simulink model "CHBPWM"  (R2022a)
settings: Solver=ode23  StartTime=0.0  StopTime=0.1  MaxStep=1e-5  RelTol=1e-3
libraries: spsDCVoltageSourceLib x1, spsThreePhaseSeriesRLCBranchLib x1, spsThreePhaseVIMeasurementLib x1, spsUniversalBridgeLib x1, spspowerguiLib x1
settings Model: Creator=123  LastModifiedBy=123

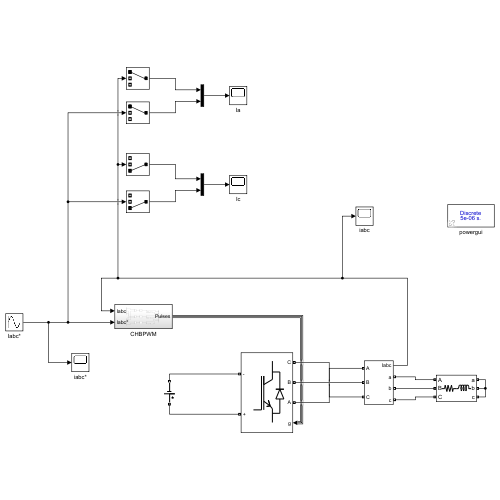
[thumbnail: Simulink's stored preview of the top-level diagram]
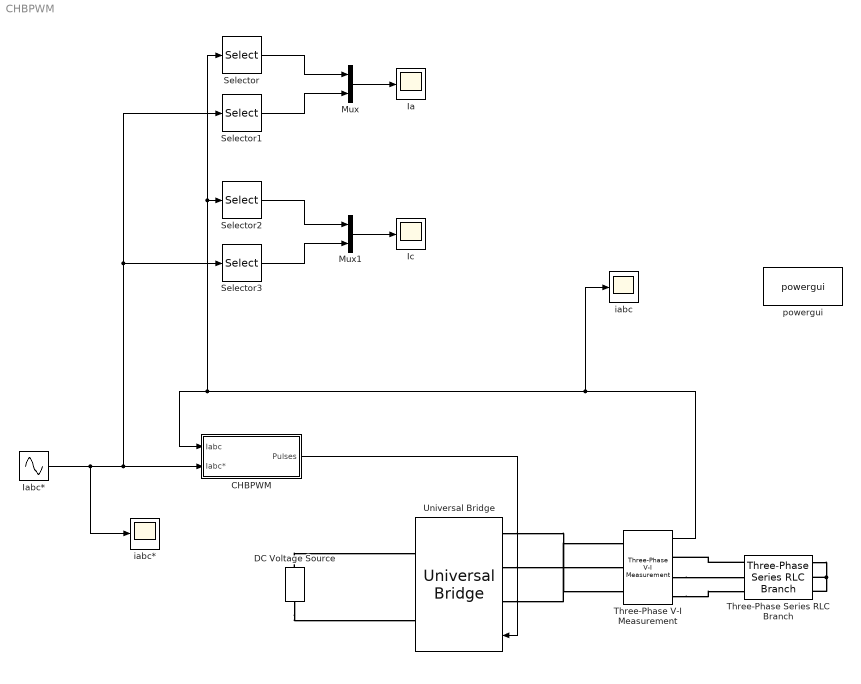
== system CHBPWM ==
  CHBPWM : Subsystem
  DC Voltage Source : spsDCVoltageSourceLib/DC Voltage Source  Amplitude=350  Measurements=None
  Ia : Scope
  Iabc* : Sin  Amplitude=10  Frequency=2*pi*50  Phase=[0,-2/3*pi,2/3*pi]  SampleTime=0
  Ic : Scope
  Mux : Mux  Inputs=2
  Mux1 : Mux  Inputs=2
  Selector : Selector  InputPortWidth=3  IndexOptions=Index vector (dialog)  Indices=[1]  OutputSizes=1
  Selector1 : Selector  InputPortWidth=3  IndexOptions=Index vector (dialog)  Indices=[1]  OutputSizes=1
  Selector2 : Selector  InputPortWidth=3  IndexOptions=Index vector (dialog)  Indices=[3]  OutputSizes=1
  Selector3 : Selector  InputPortWidth=3  IndexOptions=Index vector (dialog)  Indices=[3]  OutputSizes=1
  Three-Phase Series RLC Branch : spsThreePhaseSeriesRLCBranchLib/Three-Phase Series RLC Branch  LConnTagsString=A|B|C  RConnTagsString=A|B|C  BranchType=RL  Resistance=1  Inductance=1e-3  Capacitance=1e-6  Measurements=None
  Three-Phase V-I Measurement : spsThreePhaseVIMeasurementLib/Three-Phase V-I Measurement  VoltageMeasurement=no  SetLabelV=off  LabelV=Vabc  Vpu=off  VpuLL=off  CurrentMeasurement=yes  SetLabelI=off  LabelI=Iabc  Ipu=off  Pbase=100e6  Vbase=500e3  OutputType=Complex  PhasorSimulation=off  PSBequivalent=0
  Universal Bridge : spsUniversalBridgeLib/Universal Bridge  Arms=3  SnubberResistance=1e5  SnubberCapacitance=inf  Device=IGBT / Diodes  Ron=1e-3  Lon=0  ForwardVoltages="[  0  0  ]"  ForwardVoltage=0  GTOparameters=[ 10e-6 , 20e-6 ]  IGBTparameters=[ 1e-6 , 2e-6 ]  Measurements=None  Measurements_2=None  converterType=Rectifier
  iabc : Scope
  iabc* : Scope
  powergui : spspowerguiLib/powergui  Priority=1  SimulationMode=Discrete  SampleTime=5e-6  frequency=60  Iterations=50  frequencyindice=0  Pbase=100e6  ErrMax=1e-4  UnitsV=kV  UnitsW=MW  buscounter=0  FunctionMessages=off  echomessages=off  EnableUseOfTLC=off  CurrentSourceSwitches=off  DisableSnubberDevices=off  DisableRonSwitches=off  DisableVfSwitches=off  DisplayEquations=off  AutomaticDiscreteSolvers=off  SolverType=Tustin/Backward Euler (TBE)  Interpol=off  ExternalGateDelay=off  methode=off  Ts=100  x0status=blocks  SPID=on  SwTol=0  HookPort=off  NonlinearTolerance=1e-4  nMaxIteration=100  ContinueOnMaxIteration=off  RestoreLinks=warning  ResistiveCurrentMeasurement=off  Frange=[0:2:500]  Ylog=off  Xlog=on  ShowGrid=off  save=off  variable=ZData  structure=0  ZoomFFT=off  StartTime=0.0  cycles=1  DisplayStyle=1  fundamental=60  FreqAxis=off  MaxFrequency=1000  frequencyindicesteady=1  RmsSteady=1  display=off
  wires:
  Iabc*/1 -> Selector3/1, Selector1/1, CHBPWM/2(Iabc*), iabc*/1
  Selector/1 -> Mux/1
  Selector1/1 -> Mux/2
  Selector2/1 -> Mux1/1
  Selector3/1 -> Mux1/2
  Mux/1 -> Ia/1
  Mux1/1 -> Ic/1
  CHBPWM/1(Pulses) -> Universal Bridge/1
  Three-Phase V-I Measurement/1 -> iabc/1, Selector/1, Selector2/1, CHBPWM/1(Iabc)
  connections:
  DC Voltage Source/LConn1 -- Universal Bridge/RConn2
  DC Voltage Source/RConn1 -- Universal Bridge/RConn1
  Universal Bridge/LConn3 -- Three-Phase V-I Measurement/LConn3
  Universal Bridge/LConn2 -- Three-Phase V-I Measurement/LConn2
  Universal Bridge/LConn1 -- Three-Phase V-I Measurement/LConn1
  Three-Phase Series RLC Branch/LConn1 -- Three-Phase V-I Measurement/RConn1
  Three-Phase V-I Measurement/RConn2 -- Three-Phase Series RLC Branch/LConn2
  Three-Phase Series RLC Branch/RConn1 -- Three-Phase Series RLC Branch/RConn3 -- Three-Phase Series RLC Branch/RConn2
  Three-Phase V-I Measurement/RConn3 -- Three-Phase Series RLC Branch/LConn3

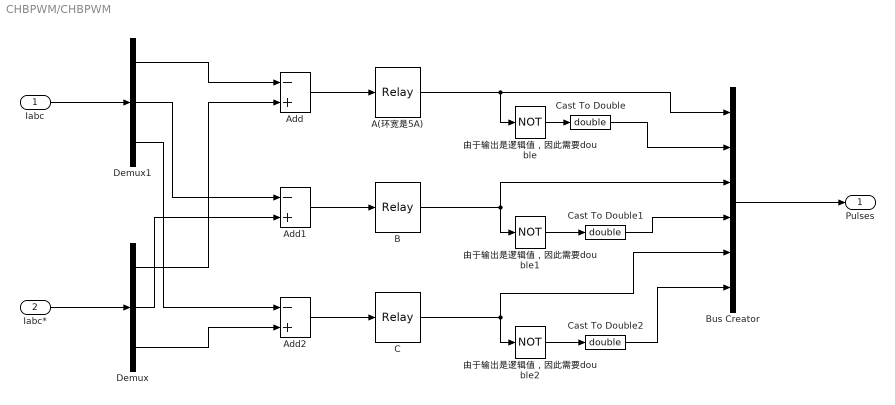
== system CHBPWM/CHBPWM ==
  Iabc : Inport
  Iabc* : Inport  Port=2
  A(环宽是5A) : Relay  OnSwitchValue=2.5  OffSwitchValue=-2.5
  Add : Sum  Inputs=-+
  Add1 : Sum  Inputs=-+
  Add2 : Sum  Inputs=-+
  B : Relay  OnSwitchValue=2.5  OffSwitchValue=-2.5
  Bus Creator : BusCreator  Inputs=6
  C : Relay  OnSwitchValue=2.5  OffSwitchValue=-2.5
  Cast To Double : DataTypeConversion  OutDataTypeStr=double  SaturateOnIntegerOverflow=off  RndMeth=Floor
  Cast To Double1 : DataTypeConversion  OutDataTypeStr=double  SaturateOnIntegerOverflow=off  RndMeth=Floor
  Cast To Double2 : DataTypeConversion  OutDataTypeStr=double  SaturateOnIntegerOverflow=off  RndMeth=Floor
  Demux : Demux  Outputs=3
  Demux1 : Demux  Outputs=3
  由于输出是逻辑值，因此需要double : Logic  Operator=NOT  AllPortsSameDT=off  OutDataTypeStr=boolean
  由于输出是逻辑值，因此需要double1 : Logic  Operator=NOT  AllPortsSameDT=off  OutDataTypeStr=boolean
  由于输出是逻辑值，因此需要double2 : Logic  Operator=NOT  AllPortsSameDT=off  OutDataTypeStr=boolean
  Pulses : Outport
  wires:
  Iabc/1 -> Demux1/1
  Iabc*/1 -> Demux/1
  Demux1/1 -> Add/1
  Demux/1 -> Add/2
  Demux1/2 -> Add1/1
  Demux/2 -> Add1/2
  Demux1/3 -> Add2/1
  Demux/3 -> Add2/2
  Add/1 -> A(环宽是5A)/1
  Add1/1 -> B/1
  Add2/1 -> C/1
  A(环宽是5A)/1 -> 由于输出是逻辑值，因此需要double/1, Bus Creator/1
  Bus Creator/1 -> Pulses/1
  B/1 -> 由于输出是逻辑值，因此需要double1/1, Bus Creator/3
  C/1 -> 由于输出是逻辑值，因此需要double2/1, Bus Creator/5
  由于输出是逻辑值，因此需要double/1 -> Cast To Double/1
  Cast To Double/1 -> Bus Creator/2
  由于输出是逻辑值，因此需要double2/1 -> Cast To Double2/1
  Cast To Double2/1 -> Bus Creator/6
  由于输出是逻辑值，因此需要double1/1 -> Cast To Double1/1
  Cast To Double1/1 -> Bus Creator/4
